simulink model "ladrc_model_dt"  (R2024a)
settings: Solver=ode4  StartTime=0.0  StopTime=10.0  FixedStep=0.001  RelTol=1e-3
values from neighbouring files (symbols this model uses):
  K = 1    [Q1_a_1.m]    (also in Q1_a_2.m; Q1_a_3.m; Q1_a_4.m; Q1_a_5.m)
  k_ob_const = 10    [Q1_a_6.m]
  T = T_values(i)    [Q1_a_1.m]    (also in Q1_a_2.m = T_values(ti); Q1_a_3.m = T_values(ti); Q1_a_4.m = 1; Q1_a_5.m = 1)
  T_dead = 0    [Q1_a_6.m]
  T_dead_ESO = 0    [Q1_a_6.m]
undefined symbols (not defined in the file or in its folder): Ts_sample
libraries: simulink x1
settings Model: Creator=Asus  LastModifiedBy=Asus

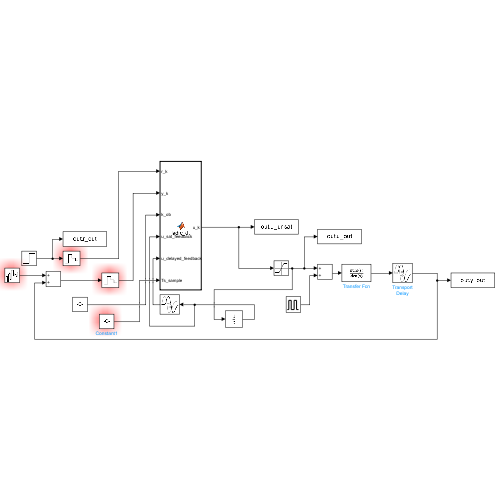
[thumbnail: Simulink's stored preview of the top-level diagram]
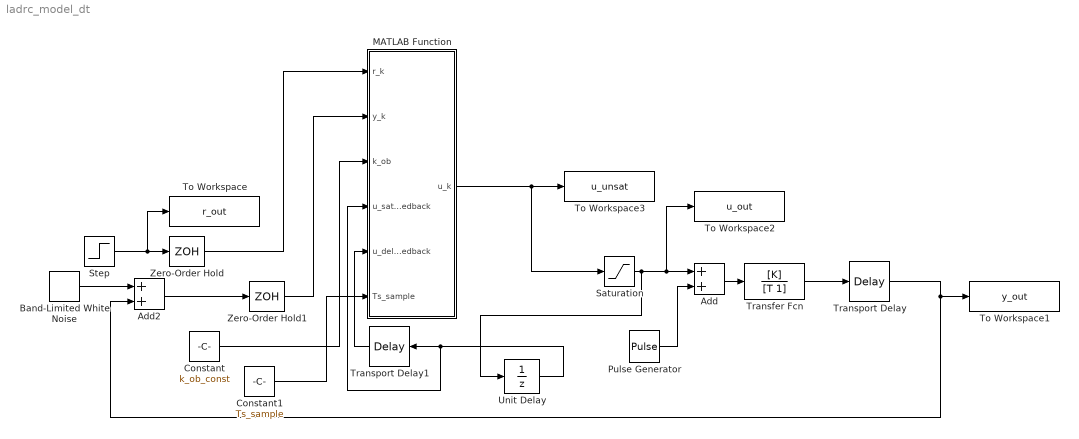
== system ladrc_model_dt ==
  Add : Sum
  Add2 : Sum
  Band-Limited White Noise : simulink/Sources/Band-Limited White Noise  Cov=noise_var  Ts=0.001  seed=[23341]
  Constant : Constant  Value=k_ob_const  SampleTime=0.001
  Constant1 : Constant  Value=Ts_sample  SampleTime=0.001
  MATLAB Function : MATLAB Function  TreatAsAtomicUnit=on  SystemSampleTime=0.001
  Pulse Generator : DiscretePulseGenerator  PulseType=Time based  PulseWidth=99  PhaseDelay=2
  Saturation : Saturate  UpperLimit=100  LowerLimit=-100
  Step : Step  Time=0  SampleTime=0
  To Workspace : ToWorkspace  VariableName=r_out  SampleTime=-1
  To Workspace1 : ToWorkspace  VariableName=y_out  SampleTime=-1
  To Workspace2 : ToWorkspace  VariableName=u_out  SampleTime=-1
  To Workspace3 : ToWorkspace  VariableName=u_unsat  SampleTime=0.001
  Transfer Fcn : TransferFcn  Numerator=[K]  Denominator=[T 1]
  Transport Delay : TransportDelay  DelayTime=T_dead
  Transport Delay1 : TransportDelay  DelayTime=T_dead_ESO
  Unit Delay : UnitDelay  SampleTime=0.001  HasFrameUpgradeWarning=on
  Zero-Order Hold : ZeroOrderHold  SampleTime=Ts_sample
  Zero-Order Hold1 : ZeroOrderHold  SampleTime=Ts_sample
  wires:
  MATLAB Function/1(u_k) -> Saturation/1, To Workspace3/1
  Step/1 -> To Workspace/1, Zero-Order Hold/1
  Zero-Order Hold/1 -> MATLAB Function/1(r_k)
  Zero-Order Hold1/1 -> MATLAB Function/2(y_k)
  Constant/1 -> MATLAB Function/3(k_ob)
  Saturation/1 -> Unit Delay/1, Add/1, To Workspace2/1
  Unit Delay/1 -> MATLAB Function/4(u_sat_feedback), Transport Delay1/1
  Transport Delay/1 -> Add2/2, To Workspace1/1
  Transport Delay1/1 -> MATLAB Function/5(u_delayed_feedback)
  Transfer Fcn/1 -> Transport Delay/1
  Pulse Generator/1 -> Add/2
  Add/1 -> Transfer Fcn/1
  Add2/1 -> Zero-Order Hold1/1
  Band-Limited White Noise/1 -> Add2/1
  Constant1/1 -> MATLAB Function/6(Ts_sample)

== matlab function ladrc_model_dt/MATLAB Function ==
  data: r_k input; u_k output; y_k input; k_ob input; u_sat_feedback input; u_delayed_feedback input; Ts_sample input
function u_k = ladrc_dt(r_k, y_k, k_ob, u_sat_feedback, u_delayed_feedback, Ts_sample)
    % tuning parameters, im writing the code for this block as following so
    % i only have to change these paramters every time 
    T_settle = 1; 
    b0 = 1; 
    Ts = Ts_sample;

    % persistent variables holding states from step (k-1)
    persistent x_hat_k_minus_1 u_k_minus_1
    if isempty(x_hat_k_minus_1)
        x_hat_k_minus_1 = [0; 0]; 
        u_k_minus_1 = 0; 
    end

    % kp , poles , L , Ad ,  Bd and cd
    Kp = 4 / T_settle; 
    s_CL = -Kp; 
    s_ESO = k_ob * s_CL;
    z_ESO = exp(s_ESO * Ts);
    
    l1 = 1 - z_ESO^2; 
    l2 = (1 / Ts) * (1 - z_ESO)^2; 
    Ld = [l1; l2];
    
    Ad = [1, Ts; 0, 1]; 
    Bd = [b0 * Ts; 0]; 
    Cd = [1, 0];
    
    % observer would calculate current estimate x_hat(k)
    x_hat_k = (Ad - Ld * Cd * Ad) * x_hat_k_minus_1 + (Bd - Ld * Cd * Bd) * u_k_minus_1 + Ld * y_k;
    
    % our control Law would calculate current output u(k) 
    u_k = (1 / b0) * (Kp * (r_k - x_hat_k(1)) - x_hat_k(2));
    
    % update Memory for next Step (Current becomes k-1 for the next
    % loop ) 
    x_hat_k_minus_1 = x_hat_k ; 
    u_k_minus_1 = u_delayed_feedback;
end
